simulink model "simulation_4_different_capacity"  (R2026a)
settings: Solver=VariableStepAuto  StopTime=12000
undefined symbols (not defined in the file): battery_builder_rtmsupport, gcbh
libraries: fl_lib x36, nesl_utility x18, BatteryCurrentManagement x6, Batteries_lib x6, BatteryEstimators x6
(part 1 of 2)
settings Model: Creator=dom  LastModifiedBy=dom

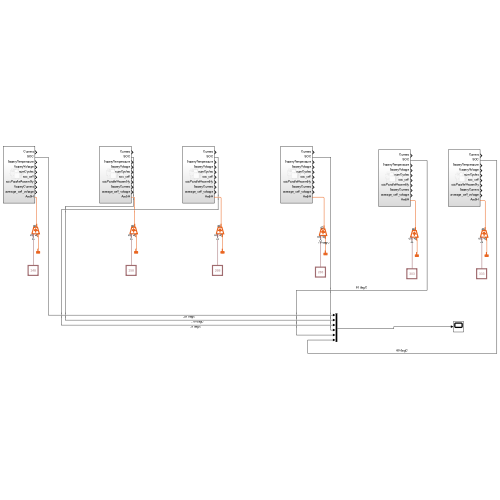
[thumbnail: Simulink's stored preview of the top-level diagram]
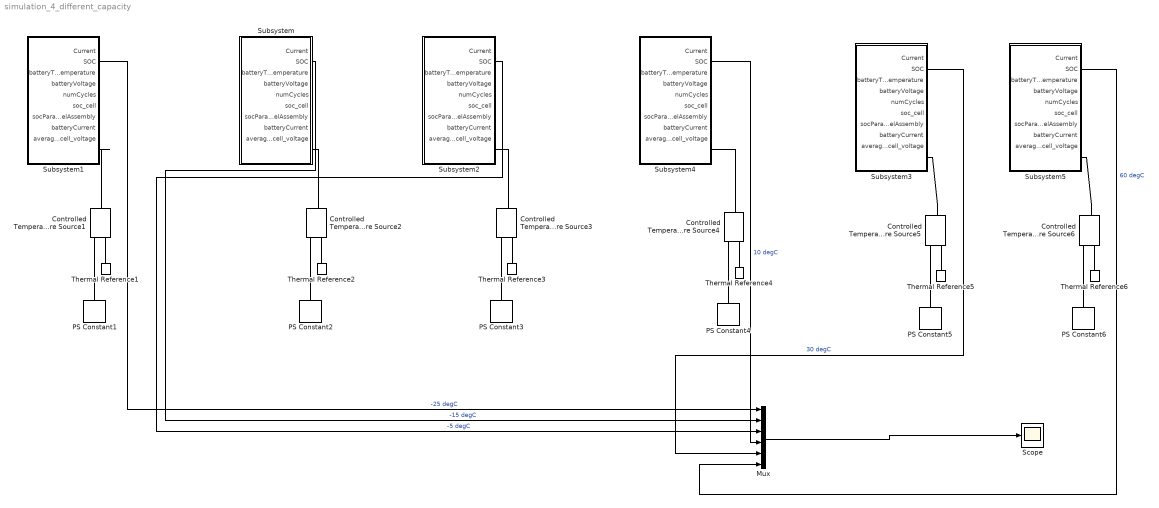
== system simulation_4_different_capacity ==
  Controlled Temperature Source{1..6} (6 alike) : fl_lib/Thermal/Thermal Sources/Controlled Temperature Source
  Mux : Mux  Inputs=6
  PS Constant1 : fl_lib/Physical Signals/Sources/PS Constant  constant=248 K
  PS Constant2 : fl_lib/Physical Signals/Sources/PS Constant  constant=258 K
  PS Constant3 : fl_lib/Physical Signals/Sources/PS Constant  constant=268 K
  PS Constant4 : fl_lib/Physical Signals/Sources/PS Constant  constant=283 K
  PS Constant5 : fl_lib/Physical Signals/Sources/PS Constant  constant=303 K
  PS Constant6 : fl_lib/Physical Signals/Sources/PS Constant  constant=333 K
  Scope : Scope
      settings: ActiveDisplayYMinimum=2.8193312500000003  ActiveDisplayYMaximum=4.3218187500000012
  Subsystem : Subsystem
  Subsystem1 : Subsystem
  Subsystem2 : Subsystem
  Subsystem3 : Subsystem
  Subsystem4 : Subsystem
  Subsystem5 : Subsystem
  Thermal Reference{1..6} (6 alike) : fl_lib/Thermal/Thermal Elements/Thermal Reference
  wires:
  Mux/1 -> Scope/1
  Subsystem1/2(SOC) -> Mux/1  "-25 degC"
  Subsystem/2(SOC) -> Mux/2  "-15 degC"
  Subsystem2/2(SOC) -> Mux/3  "-5 degC"
  Subsystem4/2(SOC) -> Mux/4  "10 degC"
  Subsystem3/2(SOC) -> Mux/5  "30 degC"
  Subsystem5/2(SOC) -> Mux/6  "60 degC"
  connections:
  PS Constant1/RConn1 -- Controlled Temperature Source1/RConn1
  Controlled Temperature Source1/RConn2 -- Thermal Reference1/LConn1
  Subsystem1/RConn1 -- Controlled Temperature Source1/LConn1
  Controlled Temperature Source2/LConn1 -- Subsystem/RConn1
  PS Constant2/RConn1 -- Controlled Temperature Source2/RConn1
  Controlled Temperature Source2/RConn2 -- Thermal Reference2/LConn1
  Controlled Temperature Source3/LConn1 -- Subsystem2/RConn1
  PS Constant3/RConn1 -- Controlled Temperature Source3/RConn1
  Controlled Temperature Source3/RConn2 -- Thermal Reference3/LConn1
  Controlled Temperature Source4/LConn1 -- Subsystem4/RConn1
  PS Constant4/RConn1 -- Controlled Temperature Source4/RConn1
  Controlled Temperature Source4/RConn2 -- Thermal Reference4/LConn1
  Controlled Temperature Source5/LConn1 -- Subsystem3/RConn1
  PS Constant5/RConn1 -- Controlled Temperature Source5/RConn1
  Controlled Temperature Source5/RConn2 -- Thermal Reference5/LConn1
  PS Constant6/RConn1 -- Controlled Temperature Source6/RConn1
  Controlled Temperature Source6/RConn2 -- Thermal Reference6/LConn1
  Controlled Temperature Source6/LConn1 -- Subsystem5/RConn1

== system simulation_4_different_capacity/Subsystem ==
  CC-CV Controller : BatteryCurrentManagement/Battery CC-CV  MinMaxFlag=off  MaxCellVoltage=4.2  Kp=100  Ki=10  Kaw=1  Kt=1  Ts=1
      settings: LibrarySourceBlock=batt_sl_lib/Current Management/Battery CC-CV
  Constant : Constant
  Constant1 : Constant  Value=10.4
  Controlled Current Source : fl_lib/Electrical/Electrical Sources/Controlled Current Source
  Current Sensor : fl_lib/Electrical/Electrical Sensors/Current Sensor
  Electrical Reference : fl_lib/Electrical/Electrical Elements/Electrical Reference
  Gain : Gain  Gain=0.5
  Gain1 : Gain  Gain=-1
  Mean : MATLAB Function  TreatAsAtomicUnit=on
  ODPC : MATLAB Function  TreatAsAtomicUnit=on
  PS-Simulink Converter : nesl_utility/PS-Simulink Converter  PhysicalDomain=network_engine_domain  SubClassName=ps_output  LeftPortType=input  RightPortType=output  PseudoPeriodic=off  Frequencies=[]  VectorFormat=inherit  Unit=inherit  AffineConversion=off
  Project_Pack : Subsystem  LoadFcn=battery_builder_rtmsupport('loadfcn',gcbh);
      settings: CopyFcn=battery_builder_rtmsupport('copyfcn',gcbh);  PreCopyFcn=battery_builder_rtmsupport('precopyfcn',gcbh);  PreDeleteFcn=battery_builder_rtmsupport('predeletefcn',gcbh);  PortSchema="{\"entries\":[{\"content\":{\"sides\":[{\"content\":{\"connectorIds\":[\"LConn1\"]},\"type\":\"ConnectorPlacement.EquallySpacedRectSide\",\"uuid\":\"76c6f046-db8e-4015-a922-00ba973faf16\"},{\"content\":{\"connectorIds\":[\"RConn1\",\"RConn2\"],\"side\":\"RIGHT\"},\"type\":\"ConnectorPlacement.EquallySpacedRectSide\",\"uuid\":\"59fdee5c-a6f4-4b44-aa6e-82d2d9418fce\"},{\"content\":{\"connectorIds\":[\"Out7\"],\"side\":\"TOP\"},\"type\":\"ConnectorPlacement.EquallySpacedRectSide\",\"uuid\":\"84b83595-cc1f-46da-a2b0-c16634a6daab\"},{\"content\":{\"connectorIds\":[\"Out1\",\"Out2\",\"Out3\",\"Out4\",\"Out5\",\"Out6\"],\"side\":\"BOTTOM\"},\"type\":\"ConnectorPlacement.EquallySpacedRectSide\",\"uuid\":\"4528fa0d-8164-4e66-baa6-2a345765de4f\"}]},\"type\":\"ConnectorPlacement.EquallySpacedConnector\",\"uuid\":\"e6fb231a-8daf-4bfc-bdc1-9175fa7a2dfd\"}],\"packageUris\":[\"http://schema.mathworks.com/mf0/Connector/R2020b\"],\"version\":\"1.0\"}"
      mask Display: image('$imagefile')
  Relay : Relay  OnSwitchValue=1  OffSwitchValue=0  OnOutputValue=0  OffOutputValue=1
  "SOC Estimator " : BatteryEstimators/SOC Estimator (Coulomb Counting)  CurrentInputPartition=off  AH=7.08  Ts=1  DataType=Inherit: auto
      settings: LibrarySourceBlock=|
      | batt_sl_lib/Estimators/SOC Estimator
      | (Coulomb Counting)
  Simulink-PS Converter1 : nesl_utility/Simulink-PS Converter  PhysicalDomain=network_engine_domain  SubClassName=ps_input  LeftPortType=input  RightPortType=output  PseudoPeriodic=off  Frequencies=[]  NoiseDistribution=none  NoiseParameters=[]  Unit=1  AffineConversion=off  FilteringAndDerivatives=provide  SimscapeFilterOrder=1  InputFilterTimeConstant=0.001  UdotUserProvided=0
  Solver Configuration : nesl_utility/Solver Configuration  PhysicalDomain=network_engine_domain  SubClassName=solver  LeftPortType=input  RightPortType=generic  Tones=[]  Harmonics=[]  SimulateNoise=off  Profile=off  UseLocalSampling=off  EnableSwitchedLinearOptims=on  FrequencyDomain=off  UseCCode=off  RelTol=0.001  AbsTol=0.001  MinStep=1e-09  ToWorkspace=off  RevertToSquareIcSolve=off  NumHomotopyIterations=100  PhasorMode=off  PhasorModeNumHarmonics=1  ConsistencySolver=NEWTON_XTOL_AFTER_FTOL  CanonicalOrdering=CANONICAL  OptimizeIntermediates=OPTIMIZED  IndexReductionMethod=DerivativeReplacement  DoDC=off  ResidualTolerance=1e-09  ConsistencyTolSource=GLOBAL  ConsistencyAbsTol=0.001  ConsistencyRelTol=0.001  ConsistencyTolFactor=0.001  UseLocalSolver=off  LocalSolverChoice=NE_BACKWARD_EULER_ADVANCER  ResolveIndetEquations=on  FunctionEvalNumThread=1  LocalSolverSampleTime=0.001  DoFixedCost=off  MaxNonlinIter=3  MaxModeIter=2  ComputeImpulses=off  ImpulseIterations=2  LinearAlgebra=auto  LinearAlgebraNumThread=0  EquationFormulation=NE_TIME_EF  DelaysMemoryBudget=1024  AutomaticFiltering=on  FilteringTimeConstant=0.001  PartitionStorageMethod=AS_NEEDED  PartitionMemoryBudget=1024  PartitionMethod=ROBUST  MultibodyUseLocalSolver=off  MultibodyLocalSolverChoice=ODE1  MultibodyLocalSolverSampleTime=0.001
  Unit Delay : UnitDelay  InitialCondition=4.2
  Unit Delay1 : UnitDelay  InitialCondition=1
  Unit Delay2 : UnitDelay  SampleTime=-1
  AmbH : PMIOPort  Side=Right
  Current : Outport
  SOC : Outport  Port=2
  batteryTemperature : Outport  Port=3
  batteryVoltage : Outport  Port=4
  numCycles : Outport  Port=5
  soc_cell : Outport  Port=6
  socParallelAssembly : Outport  Port=7
  batteryCurrent : Outport  Port=8
  average_cell_voltage : Outport  Port=9
  wires:
  Project_Pack/1(batteryTemperature) -> batteryTemperature/1  "batteryTemperature"
  CC-CV Controller/1 -> ODPC/3(CC_CV_current)
  ODPC/1(output_current) -> Simulink-PS Converter1/1  "output_current"
  Gain1/1 -> CC-CV Controller/4
  Project_Pack/3(numCycles) -> numCycles/1
  Mean/1(y) -> average_cell_voltage/1, Unit Delay/1  "average_cell_voltage"
  Project_Pack/2(batteryVoltage) -> batteryVoltage/1
  Unit Delay1/1 -> ODPC/2(SOC), Relay/1
  Unit Delay2/1 -> ODPC/1(charging_enabled)
  Constant1/1 -> Gain/1, Gain1/1  "pack_C-rate"
  Unit Delay/1 -> CC-CV Controller/2
  Project_Pack/6(batteryCurrent) -> batteryCurrent/1
  Constant/1 -> "SOC Estimator "/2
  Project_Pack/4(socCell) -> soc_cell/1  "soc_cell"
  "SOC Estimator "/1 -> SOC/1, Unit Delay1/1  "SOC"
  Project_Pack/7(vParallelAssembly) -> Mean/1(u)
  PS-Simulink Converter/1 -> Current/1, "SOC Estimator "/1
  Gain/1 -> CC-CV Controller/3
  Relay/1 -> Unit Delay2/1, CC-CV Controller/1  "charging_enabled"
  Project_Pack/5(socParallelAssembly) -> socParallelAssembly/1
  connections:
  Project_Pack/RConn1 -- AmbH/RConn1
  Controlled Current Source/LConn1 -- Project_Pack/LConn1
  Simulink-PS Converter1/RConn1 -- Controlled Current Source/RConn1
  Project_Pack/RConn2 -- Solver Configuration/RConn1 -- Current Sensor/LConn1 -- Electrical Reference/LConn1
  Current Sensor/RConn1 -- PS-Simulink Converter/LConn1
  Current Sensor/RConn2 -- Controlled Current Source/RConn2

== system simulation_4_different_capacity/Subsystem1 ==
  CC-CV Controller : BatteryCurrentManagement/Battery CC-CV  MinMaxFlag=off  MaxCellVoltage=4.2  Kp=100  Ki=10  Kaw=1  Kt=1  Ts=1
      settings: LibrarySourceBlock=batt_sl_lib/Current Management/Battery CC-CV
  Constant : Constant
  Constant1 : Constant  Value=10.4
  Controlled Current Source : fl_lib/Electrical/Electrical Sources/Controlled Current Source
  Current Sensor : fl_lib/Electrical/Electrical Sensors/Current Sensor
  Electrical Reference : fl_lib/Electrical/Electrical Elements/Electrical Reference
  Gain : Gain  Gain=0.5
  Gain1 : Gain  Gain=-1
  Mean : MATLAB Function  TreatAsAtomicUnit=on
  ODPC : MATLAB Function  TreatAsAtomicUnit=on
  PS-Simulink Converter : nesl_utility/PS-Simulink Converter  PhysicalDomain=network_engine_domain  SubClassName=ps_output  LeftPortType=input  RightPortType=output  PseudoPeriodic=off  Frequencies=[]  VectorFormat=inherit  Unit=inherit  AffineConversion=off
  Project_Pack : Subsystem  LoadFcn=battery_builder_rtmsupport('loadfcn',gcbh);
      settings: CopyFcn=battery_builder_rtmsupport('copyfcn',gcbh);  PreCopyFcn=battery_builder_rtmsupport('precopyfcn',gcbh);  PreDeleteFcn=battery_builder_rtmsupport('predeletefcn',gcbh);  PortSchema="{\"entries\":[{\"content\":{\"sides\":[{\"content\":{\"connectorIds\":[\"LConn1\"]},\"type\":\"ConnectorPlacement.EquallySpacedRectSide\",\"uuid\":\"76c6f046-db8e-4015-a922-00ba973faf16\"},{\"content\":{\"connectorIds\":[\"RConn1\",\"RConn2\"],\"side\":\"RIGHT\"},\"type\":\"ConnectorPlacement.EquallySpacedRectSide\",\"uuid\":\"59fdee5c-a6f4-4b44-aa6e-82d2d9418fce\"},{\"content\":{\"connectorIds\":[\"Out7\"],\"side\":\"TOP\"},\"type\":\"ConnectorPlacement.EquallySpacedRectSide\",\"uuid\":\"84b83595-cc1f-46da-a2b0-c16634a6daab\"},{\"content\":{\"connectorIds\":[\"Out1\",\"Out2\",\"Out3\",\"Out4\",\"Out5\",\"Out6\"],\"side\":\"BOTTOM\"},\"type\":\"ConnectorPlacement.EquallySpacedRectSide\",\"uuid\":\"4528fa0d-8164-4e66-baa6-2a345765de4f\"}]},\"type\":\"ConnectorPlacement.EquallySpacedConnector\",\"uuid\":\"e6fb231a-8daf-4bfc-bdc1-9175fa7a2dfd\"}],\"packageUris\":[\"http://schema.mathworks.com/mf0/Connector/R2020b\"],\"version\":\"1.0\"}"
      mask Display: image('$imagefile')
  Relay : Relay  OnSwitchValue=1  OffSwitchValue=0  OnOutputValue=0  OffOutputValue=1
  "SOC Estimator " : BatteryEstimators/SOC Estimator (Coulomb Counting)  CurrentInputPartition=off  AH=4.2  Ts=1  DataType=Inherit: auto
      settings: LibrarySourceBlock=|
      | batt_sl_lib/Estimators/SOC Estimator
      | (Coulomb Counting)
  Simulink-PS Converter1 : nesl_utility/Simulink-PS Converter  PhysicalDomain=network_engine_domain  SubClassName=ps_input  LeftPortType=input  RightPortType=output  PseudoPeriodic=off  Frequencies=[]  NoiseDistribution=none  NoiseParameters=[]  Unit=1  AffineConversion=off  FilteringAndDerivatives=provide  SimscapeFilterOrder=1  InputFilterTimeConstant=0.001  UdotUserProvided=0
  Solver Configuration : nesl_utility/Solver Configuration  PhysicalDomain=network_engine_domain  SubClassName=solver  LeftPortType=input  RightPortType=generic  Tones=[]  Harmonics=[]  SimulateNoise=off  Profile=off  UseLocalSampling=off  EnableSwitchedLinearOptims=on  FrequencyDomain=off  UseCCode=off  RelTol=0.001  AbsTol=0.001  MinStep=1e-09  ToWorkspace=off  RevertToSquareIcSolve=off  NumHomotopyIterations=100  PhasorMode=off  PhasorModeNumHarmonics=1  ConsistencySolver=NEWTON_XTOL_AFTER_FTOL  CanonicalOrdering=CANONICAL  OptimizeIntermediates=OPTIMIZED  IndexReductionMethod=DerivativeReplacement  DoDC=off  ResidualTolerance=1e-09  ConsistencyTolSource=GLOBAL  ConsistencyAbsTol=0.001  ConsistencyRelTol=0.001  ConsistencyTolFactor=0.001  UseLocalSolver=off  LocalSolverChoice=NE_BACKWARD_EULER_ADVANCER  ResolveIndetEquations=on  FunctionEvalNumThread=1  LocalSolverSampleTime=0.001  DoFixedCost=off  MaxNonlinIter=3  MaxModeIter=2  ComputeImpulses=off  ImpulseIterations=2  LinearAlgebra=auto  LinearAlgebraNumThread=0  EquationFormulation=NE_TIME_EF  DelaysMemoryBudget=1024  AutomaticFiltering=on  FilteringTimeConstant=0.001  PartitionStorageMethod=AS_NEEDED  PartitionMemoryBudget=1024  PartitionMethod=ROBUST  MultibodyUseLocalSolver=off  MultibodyLocalSolverChoice=ODE1  MultibodyLocalSolverSampleTime=0.001
  Unit Delay : UnitDelay  InitialCondition=4.2
  Unit Delay1 : UnitDelay  InitialCondition=1
  Unit Delay2 : UnitDelay  SampleTime=-1
  AmbH : PMIOPort  Side=Right
  Current : Outport
  SOC : Outport  Port=2
  batteryTemperature : Outport  Port=3
  batteryVoltage : Outport  Port=4
  numCycles : Outport  Port=5
  soc_cell : Outport  Port=6
  socParallelAssembly : Outport  Port=7
  batteryCurrent : Outport  Port=8
  average_cell_voltage : Outport  Port=9
  wires:
  Project_Pack/1(batteryTemperature) -> batteryTemperature/1  "batteryTemperature"
  CC-CV Controller/1 -> ODPC/3(CC_CV_current)
  ODPC/1(output_current) -> Simulink-PS Converter1/1  "output_current"
  Gain1/1 -> CC-CV Controller/4
  Project_Pack/3(numCycles) -> numCycles/1
  Mean/1(y) -> average_cell_voltage/1, Unit Delay/1  "average_cell_voltage"
  Project_Pack/2(batteryVoltage) -> batteryVoltage/1
  Unit Delay1/1 -> ODPC/2(SOC), Relay/1
  Unit Delay2/1 -> ODPC/1(charging_enabled)
  Constant1/1 -> Gain/1, Gain1/1  "pack_C-rate"
  Unit Delay/1 -> CC-CV Controller/2
  Project_Pack/6(batteryCurrent) -> batteryCurrent/1
  Constant/1 -> "SOC Estimator "/2
  Project_Pack/4(socCell) -> soc_cell/1  "soc_cell"
  "SOC Estimator "/1 -> SOC/1, Unit Delay1/1  "SOC"
  Project_Pack/7(vParallelAssembly) -> Mean/1(u)
  PS-Simulink Converter/1 -> Current/1, "SOC Estimator "/1
  Gain/1 -> CC-CV Controller/3
  Relay/1 -> Unit Delay2/1, CC-CV Controller/1  "charging_enabled"
  Project_Pack/5(socParallelAssembly) -> socParallelAssembly/1
  connections:
  Project_Pack/RConn1 -- AmbH/RConn1
  Controlled Current Source/LConn1 -- Project_Pack/LConn1
  Simulink-PS Converter1/RConn1 -- Controlled Current Source/RConn1
  Project_Pack/RConn2 -- Solver Configuration/RConn1 -- Current Sensor/LConn1 -- Electrical Reference/LConn1
  Current Sensor/RConn1 -- PS-Simulink Converter/LConn1
  Current Sensor/RConn2 -- Controlled Current Source/RConn2

== system simulation_4_different_capacity/Subsystem2 ==
  CC-CV Controller : BatteryCurrentManagement/Battery CC-CV  MinMaxFlag=off  MaxCellVoltage=4.2  Kp=100  Ki=10  Kaw=1  Kt=1  Ts=1
      settings: LibrarySourceBlock=batt_sl_lib/Current Management/Battery CC-CV
  Constant : Constant
  Constant1 : Constant  Value=10.4
  Controlled Current Source : fl_lib/Electrical/Electrical Sources/Controlled Current Source
  Current Sensor : fl_lib/Electrical/Electrical Sensors/Current Sensor
  Electrical Reference : fl_lib/Electrical/Electrical Elements/Electrical Reference
  Gain : Gain  Gain=0.5
  Gain1 : Gain  Gain=-1
  Mean : MATLAB Function  TreatAsAtomicUnit=on
  ODPC : MATLAB Function  TreatAsAtomicUnit=on
  PS-Simulink Converter : nesl_utility/PS-Simulink Converter  PhysicalDomain=network_engine_domain  SubClassName=ps_output  LeftPortType=input  RightPortType=output  PseudoPeriodic=off  Frequencies=[]  VectorFormat=inherit  Unit=inherit  AffineConversion=off
  Project_Pack : Subsystem  LoadFcn=battery_builder_rtmsupport('loadfcn',gcbh);
      settings: CopyFcn=battery_builder_rtmsupport('copyfcn',gcbh);  PreCopyFcn=battery_builder_rtmsupport('precopyfcn',gcbh);  PreDeleteFcn=battery_builder_rtmsupport('predeletefcn',gcbh);  PortSchema="{\"entries\":[{\"content\":{\"sides\":[{\"content\":{\"connectorIds\":[\"LConn1\"]},\"type\":\"ConnectorPlacement.EquallySpacedRectSide\",\"uuid\":\"76c6f046-db8e-4015-a922-00ba973faf16\"},{\"content\":{\"connectorIds\":[\"RConn1\",\"RConn2\"],\"side\":\"RIGHT\"},\"type\":\"ConnectorPlacement.EquallySpacedRectSide\",\"uuid\":\"59fdee5c-a6f4-4b44-aa6e-82d2d9418fce\"},{\"content\":{\"connectorIds\":[\"Out7\"],\"side\":\"TOP\"},\"type\":\"ConnectorPlacement.EquallySpacedRectSide\",\"uuid\":\"84b83595-cc1f-46da-a2b0-c16634a6daab\"},{\"content\":{\"connectorIds\":[\"Out1\",\"Out2\",\"Out3\",\"Out4\",\"Out5\",\"Out6\"],\"side\":\"BOTTOM\"},\"type\":\"ConnectorPlacement.EquallySpacedRectSide\",\"uuid\":\"4528fa0d-8164-4e66-baa6-2a345765de4f\"}]},\"type\":\"ConnectorPlacement.EquallySpacedConnector\",\"uuid\":\"e6fb231a-8daf-4bfc-bdc1-9175fa7a2dfd\"}],\"packageUris\":[\"http://schema.mathworks.com/mf0/Connector/R2020b\"],\"version\":\"1.0\"}"
      mask Display: image('$imagefile')
  Relay : Relay  OnSwitchValue=1  OffSwitchValue=0  OnOutputValue=0  OffOutputValue=1
  "SOC Estimator " : BatteryEstimators/SOC Estimator (Coulomb Counting)  CurrentInputPartition=off  AH=9.20  Ts=1  DataType=Inherit: auto
      settings: LibrarySourceBlock=|
      | batt_sl_lib/Estimators/SOC Estimator
      | (Coulomb Counting)
  Simulink-PS Converter1 : nesl_utility/Simulink-PS Converter  PhysicalDomain=network_engine_domain  SubClassName=ps_input  LeftPortType=input  RightPortType=output  PseudoPeriodic=off  Frequencies=[]  NoiseDistribution=none  NoiseParameters=[]  Unit=1  AffineConversion=off  FilteringAndDerivatives=provide  SimscapeFilterOrder=1  InputFilterTimeConstant=0.001  UdotUserProvided=0
  Solver Configuration : nesl_utility/Solver Configuration  PhysicalDomain=network_engine_domain  SubClassName=solver  LeftPortType=input  RightPortType=generic  Tones=[]  Harmonics=[]  SimulateNoise=off  Profile=off  UseLocalSampling=off  EnableSwitchedLinearOptims=on  FrequencyDomain=off  UseCCode=off  RelTol=0.001  AbsTol=0.001  MinStep=1e-09  ToWorkspace=off  RevertToSquareIcSolve=off  NumHomotopyIterations=100  PhasorMode=off  PhasorModeNumHarmonics=1  ConsistencySolver=NEWTON_XTOL_AFTER_FTOL  CanonicalOrdering=CANONICAL  OptimizeIntermediates=OPTIMIZED  IndexReductionMethod=DerivativeReplacement  DoDC=off  ResidualTolerance=1e-09  ConsistencyTolSource=GLOBAL  ConsistencyAbsTol=0.001  ConsistencyRelTol=0.001  ConsistencyTolFactor=0.001  UseLocalSolver=off  LocalSolverChoice=NE_BACKWARD_EULER_ADVANCER  ResolveIndetEquations=on  FunctionEvalNumThread=1  LocalSolverSampleTime=0.001  DoFixedCost=off  MaxNonlinIter=3  MaxModeIter=2  ComputeImpulses=off  ImpulseIterations=2  LinearAlgebra=auto  LinearAlgebraNumThread=0  EquationFormulation=NE_TIME_EF  DelaysMemoryBudget=1024  AutomaticFiltering=on  FilteringTimeConstant=0.001  PartitionStorageMethod=AS_NEEDED  PartitionMemoryBudget=1024  PartitionMethod=ROBUST  MultibodyUseLocalSolver=off  MultibodyLocalSolverChoice=ODE1  MultibodyLocalSolverSampleTime=0.001
  Unit Delay : UnitDelay  InitialCondition=4.2
  Unit Delay1 : UnitDelay  InitialCondition=1
  Unit Delay2 : UnitDelay  SampleTime=-1
  AmbH : PMIOPort  Side=Right
  Current : Outport
  SOC : Outport  Port=2
  batteryTemperature : Outport  Port=3
  batteryVoltage : Outport  Port=4
  numCycles : Outport  Port=5
  soc_cell : Outport  Port=6
  socParallelAssembly : Outport  Port=7
  batteryCurrent : Outport  Port=8
  average_cell_voltage : Outport  Port=9
  wires:
  Project_Pack/1(batteryTemperature) -> batteryTemperature/1  "batteryTemperature"
  CC-CV Controller/1 -> ODPC/3(CC_CV_current)
  ODPC/1(output_current) -> Simulink-PS Converter1/1  "output_current"
  Gain1/1 -> CC-CV Controller/4
  Project_Pack/3(numCycles) -> numCycles/1
  Mean/1(y) -> average_cell_voltage/1, Unit Delay/1  "average_cell_voltage"
  Project_Pack/2(batteryVoltage) -> batteryVoltage/1
  Unit Delay1/1 -> ODPC/2(SOC), Relay/1
  Unit Delay2/1 -> ODPC/1(charging_enabled)
  Constant1/1 -> Gain/1, Gain1/1  "pack_C-rate"
  Unit Delay/1 -> CC-CV Controller/2
  Project_Pack/6(batteryCurrent) -> batteryCurrent/1
  Constant/1 -> "SOC Estimator "/2
  Project_Pack/4(socCell) -> soc_cell/1  "soc_cell"
  "SOC Estimator "/1 -> SOC/1, Unit Delay1/1  "SOC"
  Project_Pack/7(vParallelAssembly) -> Mean/1(u)
  PS-Simulink Converter/1 -> Current/1, "SOC Estimator "/1
  Gain/1 -> CC-CV Controller/3
  Relay/1 -> Unit Delay2/1, CC-CV Controller/1  "charging_enabled"
  Project_Pack/5(socParallelAssembly) -> socParallelAssembly/1
  connections:
  Project_Pack/RConn1 -- AmbH/RConn1
  Controlled Current Source/LConn1 -- Project_Pack/LConn1
  Simulink-PS Converter1/RConn1 -- Controlled Current Source/RConn1
  Project_Pack/RConn2 -- Solver Configuration/RConn1 -- Current Sensor/LConn1 -- Electrical Reference/LConn1
  Current Sensor/RConn1 -- PS-Simulink Converter/LConn1
  Current Sensor/RConn2 -- Controlled Current Source/RConn2

== system simulation_4_different_capacity/Subsystem3 ==
  CC-CV Controller : BatteryCurrentManagement/Battery CC-CV  MinMaxFlag=off  MaxCellVoltage=4.2  Kp=100  Ki=10  Kaw=1  Kt=1  Ts=1
      settings: LibrarySourceBlock=batt_sl_lib/Current Management/Battery CC-CV
  Constant : Constant
  Constant1 : Constant  Value=10.4
  Controlled Current Source : fl_lib/Electrical/Electrical Sources/Controlled Current Source
  Current Sensor : fl_lib/Electrical/Electrical Sensors/Current Sensor
  Electrical Reference : fl_lib/Electrical/Electrical Elements/Electrical Reference
  Gain : Gain  Gain=0.5
  Gain1 : Gain  Gain=-1
  Mean : MATLAB Function  TreatAsAtomicUnit=on
  ODPC : MATLAB Function  TreatAsAtomicUnit=on
  PS-Simulink Converter : nesl_utility/PS-Simulink Converter  PhysicalDomain=network_engine_domain  SubClassName=ps_output  LeftPortType=input  RightPortType=output  PseudoPeriodic=off  Frequencies=[]  VectorFormat=inherit  Unit=inherit  AffineConversion=off
  Project_Pack : Subsystem  LoadFcn=battery_builder_rtmsupport('loadfcn',gcbh);
      settings: CopyFcn=battery_builder_rtmsupport('copyfcn',gcbh);  PreCopyFcn=battery_builder_rtmsupport('precopyfcn',gcbh);  PreDeleteFcn=battery_builder_rtmsupport('predeletefcn',gcbh);  PortSchema="{\"entries\":[{\"content\":{\"sides\":[{\"content\":{\"connectorIds\":[\"LConn1\"]},\"type\":\"ConnectorPlacement.EquallySpacedRectSide\",\"uuid\":\"76c6f046-db8e-4015-a922-00ba973faf16\"},{\"content\":{\"connectorIds\":[\"RConn1\",\"RConn2\"],\"side\":\"RIGHT\"},\"type\":\"ConnectorPlacement.EquallySpacedRectSide\",\"uuid\":\"59fdee5c-a6f4-4b44-aa6e-82d2d9418fce\"},{\"content\":{\"connectorIds\":[\"Out7\"],\"side\":\"TOP\"},\"type\":\"ConnectorPlacement.EquallySpacedRectSide\",\"uuid\":\"84b83595-cc1f-46da-a2b0-c16634a6daab\"},{\"content\":{\"connectorIds\":[\"Out1\",\"Out2\",\"Out3\",\"Out4\",\"Out5\",\"Out6\"],\"side\":\"BOTTOM\"},\"type\":\"ConnectorPlacement.EquallySpacedRectSide\",\"uuid\":\"4528fa0d-8164-4e66-baa6-2a345765de4f\"}]},\"type\":\"ConnectorPlacement.EquallySpacedConnector\",\"uuid\":\"e6fb231a-8daf-4bfc-bdc1-9175fa7a2dfd\"}],\"packageUris\":[\"http://schema.mathworks.com/mf0/Connector/R2020b\"],\"version\":\"1.0\"}"
      mask Display: image('$imagefile')
  Relay : Relay  OnSwitchValue=1  OffSwitchValue=0  OnOutputValue=0  OffOutputValue=1
  "SOC Estimator " : BatteryEstimators/SOC Estimator (Coulomb Counting)  CurrentInputPartition=off  AH=10.4  Ts=1  DataType=Inherit: auto
      settings: LibrarySourceBlock=|
      | batt_sl_lib/Estimators/SOC Estimator
      | (Coulomb Counting)
  Simulink-PS Converter1 : nesl_utility/Simulink-PS Converter  PhysicalDomain=network_engine_domain  SubClassName=ps_input  LeftPortType=input  RightPortType=output  PseudoPeriodic=off  Frequencies=[]  NoiseDistribution=none  NoiseParameters=[]  Unit=1  AffineConversion=off  FilteringAndDerivatives=provide  SimscapeFilterOrder=1  InputFilterTimeConstant=0.001  UdotUserProvided=0
  Solver Configuration : nesl_utility/Solver Configuration  PhysicalDomain=network_engine_domain  SubClassName=solver  LeftPortType=input  RightPortType=generic  Tones=[]  Harmonics=[]  SimulateNoise=off  Profile=off  UseLocalSampling=off  EnableSwitchedLinearOptims=on  FrequencyDomain=off  UseCCode=off  RelTol=0.001  AbsTol=0.001  MinStep=1e-09  ToWorkspace=off  RevertToSquareIcSolve=off  NumHomotopyIterations=100  PhasorMode=off  PhasorModeNumHarmonics=1  ConsistencySolver=NEWTON_XTOL_AFTER_FTOL  CanonicalOrdering=CANONICAL  OptimizeIntermediates=OPTIMIZED  IndexReductionMethod=DerivativeReplacement  DoDC=off  ResidualTolerance=1e-09  ConsistencyTolSource=GLOBAL  ConsistencyAbsTol=0.001  ConsistencyRelTol=0.001  ConsistencyTolFactor=0.001  UseLocalSolver=off  LocalSolverChoice=NE_BACKWARD_EULER_ADVANCER  ResolveIndetEquations=on  FunctionEvalNumThread=1  LocalSolverSampleTime=0.001  DoFixedCost=off  MaxNonlinIter=3  MaxModeIter=2  ComputeImpulses=off  ImpulseIterations=2  LinearAlgebra=auto  LinearAlgebraNumThread=0  EquationFormulation=NE_TIME_EF  DelaysMemoryBudget=1024  AutomaticFiltering=on  FilteringTimeConstant=0.001  PartitionStorageMethod=AS_NEEDED  PartitionMemoryBudget=1024  PartitionMethod=ROBUST  MultibodyUseLocalSolver=off  MultibodyLocalSolverChoice=ODE1  MultibodyLocalSolverSampleTime=0.001
  Unit Delay : UnitDelay  InitialCondition=4.2
  Unit Delay1 : UnitDelay  InitialCondition=1
  Unit Delay2 : UnitDelay  SampleTime=-1
  AmbH : PMIOPort  Side=Right
  Current : Outport
  SOC : Outport  Port=2
  batteryTemperature : Outport  Port=3
  batteryVoltage : Outport  Port=4
  numCycles : Outport  Port=5
  soc_cell : Outport  Port=6
  socParallelAssembly : Outport  Port=7
  batteryCurrent : Outport  Port=8
  average_cell_voltage : Outport  Port=9
  wires:
  Project_Pack/1(batteryTemperature) -> batteryTemperature/1  "batteryTemperature"
  CC-CV Controller/1 -> ODPC/3(CC_CV_current)
  ODPC/1(output_current) -> Simulink-PS Converter1/1  "output_current"
  Gain1/1 -> CC-CV Controller/4
  Project_Pack/3(numCycles) -> numCycles/1
  Mean/1(y) -> average_cell_voltage/1, Unit Delay/1  "average_cell_voltage"
  Project_Pack/2(batteryVoltage) -> batteryVoltage/1
  Unit Delay1/1 -> ODPC/2(SOC), Relay/1
  Unit Delay2/1 -> ODPC/1(charging_enabled)
  Constant1/1 -> Gain/1, Gain1/1  "pack_C-rate"
  Unit Delay/1 -> CC-CV Controller/2
  Project_Pack/6(batteryCurrent) -> batteryCurrent/1
  Constant/1 -> "SOC Estimator "/2
  Project_Pack/4(socCell) -> soc_cell/1  "soc_cell"
  "SOC Estimator "/1 -> SOC/1, Unit Delay1/1  "SOC"
  Project_Pack/7(vParallelAssembly) -> Mean/1(u)
  PS-Simulink Converter/1 -> Current/1, "SOC Estimator "/1
  Gain/1 -> CC-CV Controller/3
  Relay/1 -> Unit Delay2/1, CC-CV Controller/1  "charging_enabled"
  Project_Pack/5(socParallelAssembly) -> socParallelAssembly/1
  connections:
  Project_Pack/RConn1 -- AmbH/RConn1
  Controlled Current Source/LConn1 -- Project_Pack/LConn1
  Simulink-PS Converter1/RConn1 -- Controlled Current Source/RConn1
  Project_Pack/RConn2 -- Solver Configuration/RConn1 -- Current Sensor/LConn1 -- Electrical Reference/LConn1
  Current Sensor/RConn1 -- PS-Simulink Converter/LConn1
  Current Sensor/RConn2 -- Controlled Current Source/RConn2

== system simulation_4_different_capacity/Subsystem4 ==
  CC-CV Controller : BatteryCurrentManagement/Battery CC-CV  MinMaxFlag=off  MaxCellVoltage=4.2  Kp=100  Ki=10  Kaw=1  Kt=1  Ts=1
      settings: LibrarySourceBlock=batt_sl_lib/Current Management/Battery CC-CV
  Constant : Constant
  Constant1 : Constant  Value=10.4
  Controlled Current Source : fl_lib/Electrical/Electrical Sources/Controlled Current Source
  Current Sensor : fl_lib/Electrical/Electrical Sensors/Current Sensor
  Electrical Reference : fl_lib/Electrical/Electrical Elements/Electrical Reference
  Gain : Gain  Gain=0.5
  Gain1 : Gain  Gain=-1
  Mean : MATLAB Function  TreatAsAtomicUnit=on
  ODPC : MATLAB Function  TreatAsAtomicUnit=on
  PS-Simulink Converter : nesl_utility/PS-Simulink Converter  PhysicalDomain=network_engine_domain  SubClassName=ps_output  LeftPortType=input  RightPortType=output  PseudoPeriodic=off  Frequencies=[]  VectorFormat=inherit  Unit=inherit  AffineConversion=off
  Project_Pack : Subsystem  LoadFcn=battery_builder_rtmsupport('loadfcn',gcbh);
      settings: CopyFcn=battery_builder_rtmsupport('copyfcn',gcbh);  PreCopyFcn=battery_builder_rtmsupport('precopyfcn',gcbh);  PreDeleteFcn=battery_builder_rtmsupport('predeletefcn',gcbh);  PortSchema="{\"entries\":[{\"content\":{\"sides\":[{\"content\":{\"connectorIds\":[\"LConn1\"]},\"type\":\"ConnectorPlacement.EquallySpacedRectSide\",\"uuid\":\"76c6f046-db8e-4015-a922-00ba973faf16\"},{\"content\":{\"connectorIds\":[\"RConn1\",\"RConn2\"],\"side\":\"RIGHT\"},\"type\":\"ConnectorPlacement.EquallySpacedRectSide\",\"uuid\":\"59fdee5c-a6f4-4b44-aa6e-82d2d9418fce\"},{\"content\":{\"connectorIds\":[\"Out7\"],\"side\":\"TOP\"},\"type\":\"ConnectorPlacement.EquallySpacedRectSide\",\"uuid\":\"84b83595-cc1f-46da-a2b0-c16634a6daab\"},{\"content\":{\"connectorIds\":[\"Out1\",\"Out2\",\"Out3\",\"Out4\",\"Out5\",\"Out6\"],\"side\":\"BOTTOM\"},\"type\":\"ConnectorPlacement.EquallySpacedRectSide\",\"uuid\":\"4528fa0d-8164-4e66-baa6-2a345765de4f\"}]},\"type\":\"ConnectorPlacement.EquallySpacedConnector\",\"uuid\":\"e6fb231a-8daf-4bfc-bdc1-9175fa7a2dfd\"}],\"packageUris\":[\"http://schema.mathworks.com/mf0/Connector/R2020b\"],\"version\":\"1.0\"}"
      mask Display: image('$imagefile')
  Relay : Relay  OnSwitchValue=1  OffSwitchValue=0  OnOutputValue=0  OffOutputValue=1
  "SOC Estimator " : BatteryEstimators/SOC Estimator (Coulomb Counting)  CurrentInputPartition=off  AH=10.0  Ts=1  DataType=Inherit: auto
      settings: LibrarySourceBlock=|
      | batt_sl_lib/Estimators/SOC Estimator
      | (Coulomb Counting)
  Simulink-PS Converter1 : nesl_utility/Simulink-PS Converter  PhysicalDomain=network_engine_domain  SubClassName=ps_input  LeftPortType=input  RightPortType=output  PseudoPeriodic=off  Frequencies=[]  NoiseDistribution=none  NoiseParameters=[]  Unit=1  AffineConversion=off  FilteringAndDerivatives=provide  SimscapeFilterOrder=1  InputFilterTimeConstant=0.001  UdotUserProvided=0
  Solver Configuration : nesl_utility/Solver Configuration  PhysicalDomain=network_engine_domain  SubClassName=solver  LeftPortType=input  RightPortType=generic  Tones=[]  Harmonics=[]  SimulateNoise=off  Profile=off  UseLocalSampling=off  EnableSwitchedLinearOptims=on  FrequencyDomain=off  UseCCode=off  RelTol=0.001  AbsTol=0.001  MinStep=1e-09  ToWorkspace=off  RevertToSquareIcSolve=off  NumHomotopyIterations=100  PhasorMode=off  PhasorModeNumHarmonics=1  ConsistencySolver=NEWTON_XTOL_AFTER_FTOL  CanonicalOrdering=CANONICAL  OptimizeIntermediates=OPTIMIZED  IndexReductionMethod=DerivativeReplacement  DoDC=off  ResidualTolerance=1e-09  ConsistencyTolSource=GLOBAL  ConsistencyAbsTol=0.001  ConsistencyRelTol=0.001  ConsistencyTolFactor=0.001  UseLocalSolver=off  LocalSolverChoice=NE_BACKWARD_EULER_ADVANCER  ResolveIndetEquations=on  FunctionEvalNumThread=1  LocalSolverSampleTime=0.001  DoFixedCost=off  MaxNonlinIter=3  MaxModeIter=2  ComputeImpulses=off  ImpulseIterations=2  LinearAlgebra=auto  LinearAlgebraNumThread=0  EquationFormulation=NE_TIME_EF  DelaysMemoryBudget=1024  AutomaticFiltering=on  FilteringTimeConstant=0.001  PartitionStorageMethod=AS_NEEDED  PartitionMemoryBudget=1024  PartitionMethod=ROBUST  MultibodyUseLocalSolver=off  MultibodyLocalSolverChoice=ODE1  MultibodyLocalSolverSampleTime=0.001
  Unit Delay : UnitDelay  InitialCondition=4.2
  Unit Delay1 : UnitDelay  InitialCondition=1
  Unit Delay2 : UnitDelay  SampleTime=-1
  AmbH : PMIOPort  Side=Right
  Current : Outport
  SOC : Outport  Port=2
  batteryTemperature : Outport  Port=3
  batteryVoltage : Outport  Port=4
  numCycles : Outport  Port=5
  soc_cell : Outport  Port=6
  socParallelAssembly : Outport  Port=7
  batteryCurrent : Outport  Port=8
  average_cell_voltage : Outport  Port=9
  wires:
  Project_Pack/1(batteryTemperature) -> batteryTemperature/1  "batteryTemperature"
  CC-CV Controller/1 -> ODPC/3(CC_CV_current)
  ODPC/1(output_current) -> Simulink-PS Converter1/1  "output_current"
  Gain1/1 -> CC-CV Controller/4
  Project_Pack/3(numCycles) -> numCycles/1
  Mean/1(y) -> average_cell_voltage/1, Unit Delay/1  "average_cell_voltage"
  Project_Pack/2(batteryVoltage) -> batteryVoltage/1
  Unit Delay1/1 -> ODPC/2(SOC), Relay/1
  Unit Delay2/1 -> ODPC/1(charging_enabled)
  Constant1/1 -> Gain/1, Gain1/1  "pack_C-rate"
  Unit Delay/1 -> CC-CV Controller/2
  Project_Pack/6(batteryCurrent) -> batteryCurrent/1
  Constant/1 -> "SOC Estimator "/2
  Project_Pack/4(socCell) -> soc_cell/1  "soc_cell"
  "SOC Estimator "/1 -> SOC/1, Unit Delay1/1  "SOC"
  Project_Pack/7(vParallelAssembly) -> Mean/1(u)
  PS-Simulink Converter/1 -> Current/1, "SOC Estimator "/1
  Gain/1 -> CC-CV Controller/3
  Relay/1 -> Unit Delay2/1, CC-CV Controller/1  "charging_enabled"
  Project_Pack/5(socParallelAssembly) -> socParallelAssembly/1
  connections:
  Project_Pack/RConn1 -- AmbH/RConn1
  Controlled Current Source/LConn1 -- Project_Pack/LConn1
  Simulink-PS Converter1/RConn1 -- Controlled Current Source/RConn1
  Project_Pack/RConn2 -- Solver Configuration/RConn1 -- Current Sensor/LConn1 -- Electrical Reference/LConn1
  Current Sensor/RConn1 -- PS-Simulink Converter/LConn1
  Current Sensor/RConn2 -- Controlled Current Source/RConn2

== system simulation_4_different_capacity/Subsystem5 ==
  CC-CV Controller : BatteryCurrentManagement/Battery CC-CV  MinMaxFlag=off  MaxCellVoltage=4.2  Kp=100  Ki=10  Kaw=1  Kt=1  Ts=1
      settings: LibrarySourceBlock=batt_sl_lib/Current Management/Battery CC-CV
  Constant : Constant
  Constant1 : Constant  Value=10.4
  Controlled Current Source : fl_lib/Electrical/Electrical Sources/Controlled Current Source
  Current Sensor : fl_lib/Electrical/Electrical Sensors/Current Sensor
  Electrical Reference : fl_lib/Electrical/Electrical Elements/Electrical Reference
  Gain : Gain  Gain=0.5
  Gain1 : Gain  Gain=-1
  Mean : MATLAB Function  TreatAsAtomicUnit=on
  ODPC : MATLAB Function  TreatAsAtomicUnit=on
  PS-Simulink Converter : nesl_utility/PS-Simulink Converter  PhysicalDomain=network_engine_domain  SubClassName=ps_output  LeftPortType=input  RightPortType=output  PseudoPeriodic=off  Frequencies=[]  VectorFormat=inherit  Unit=inherit  AffineConversion=off
  Project_Pack : Subsystem  LoadFcn=battery_builder_rtmsupport('loadfcn',gcbh);
      settings: CopyFcn=battery_builder_rtmsupport('copyfcn',gcbh);  PreCopyFcn=battery_builder_rtmsupport('precopyfcn',gcbh);  PreDeleteFcn=battery_builder_rtmsupport('predeletefcn',gcbh);  PortSchema="{\"entries\":[{\"content\":{\"sides\":[{\"content\":{\"connectorIds\":[\"LConn1\"]},\"type\":\"ConnectorPlacement.EquallySpacedRectSide\",\"uuid\":\"76c6f046-db8e-4015-a922-00ba973faf16\"},{\"content\":{\"connectorIds\":[\"RConn1\",\"RConn2\"],\"side\":\"RIGHT\"},\"type\":\"ConnectorPlacement.EquallySpacedRectSide\",\"uuid\":\"59fdee5c-a6f4-4b44-aa6e-82d2d9418fce\"},{\"content\":{\"connectorIds\":[\"Out7\"],\"side\":\"TOP\"},\"type\":\"ConnectorPlacement.EquallySpacedRectSide\",\"uuid\":\"84b83595-cc1f-46da-a2b0-c16634a6daab\"},{\"content\":{\"connectorIds\":[\"Out1\",\"Out2\",\"Out3\",\"Out4\",\"Out5\",\"Out6\"],\"side\":\"BOTTOM\"},\"type\":\"ConnectorPlacement.EquallySpacedRectSide\",\"uuid\":\"4528fa0d-8164-4e66-baa6-2a345765de4f\"}]},\"type\":\"ConnectorPlacement.EquallySpacedConnector\",\"uuid\":\"e6fb231a-8daf-4bfc-bdc1-9175fa7a2dfd\"}],\"packageUris\":[\"http://schema.mathworks.com/mf0/Connector/R2020b\"],\"version\":\"1.0\"}"
      mask Display: image('$imagefile')
  Relay : Relay  OnSwitchValue=1  OffSwitchValue=0  OnOutputValue=0  OffOutputValue=1
  "SOC Estimator " : BatteryEstimators/SOC Estimator (Coulomb Counting)  CurrentInputPartition=off  AH=10.52  Ts=1  DataType=Inherit: auto
      settings: LibrarySourceBlock=|
      | batt_sl_lib/Estimators/SOC Estimator
      | (Coulomb Counting)
  Simulink-PS Converter1 : nesl_utility/Simulink-PS Converter  PhysicalDomain=network_engine_domain  SubClassName=ps_input  LeftPortType=input  RightPortType=output  PseudoPeriodic=off  Frequencies=[]  NoiseDistribution=none  NoiseParameters=[]  Unit=1  AffineConversion=off  FilteringAndDerivatives=provide  SimscapeFilterOrder=1  InputFilterTimeConstant=0.001  UdotUserProvided=0
  Solver Configuration : nesl_utility/Solver Configuration  PhysicalDomain=network_engine_domain  SubClassName=solver  LeftPortType=input  RightPortType=generic  Tones=[]  Harmonics=[]  SimulateNoise=off  Profile=off  UseLocalSampling=off  EnableSwitchedLinearOptims=on  FrequencyDomain=off  UseCCode=off  RelTol=0.001  AbsTol=0.001  MinStep=1e-09  ToWorkspace=off  RevertToSquareIcSolve=off  NumHomotopyIterations=100  PhasorMode=off  PhasorModeNumHarmonics=1  ConsistencySolver=NEWTON_XTOL_AFTER_FTOL  CanonicalOrdering=CANONICAL  OptimizeIntermediates=OPTIMIZED  IndexReductionMethod=DerivativeReplacement  DoDC=off  ResidualTolerance=1e-09  ConsistencyTolSource=GLOBAL  ConsistencyAbsTol=0.001  ConsistencyRelTol=0.001  ConsistencyTolFactor=0.001  UseLocalSolver=off  LocalSolverChoice=NE_BACKWARD_EULER_ADVANCER  ResolveIndetEquations=on  FunctionEvalNumThread=1  LocalSolverSampleTime=0.001  DoFixedCost=off  MaxNonlinIter=3  MaxModeIter=2  ComputeImpulses=off  ImpulseIterations=2  LinearAlgebra=auto  LinearAlgebraNumThread=0  EquationFormulation=NE_TIME_EF  DelaysMemoryBudget=1024  AutomaticFiltering=on  FilteringTimeConstant=0.001  PartitionStorageMethod=AS_NEEDED  PartitionMemoryBudget=1024  PartitionMethod=ROBUST  MultibodyUseLocalSolver=off  MultibodyLocalSolverChoice=ODE1  MultibodyLocalSolverSampleTime=0.001
  Unit Delay : UnitDelay  InitialCondition=4.2
  Unit Delay1 : UnitDelay  InitialCondition=1
  Unit Delay2 : UnitDelay  SampleTime=-1
  AmbH : PMIOPort  Side=Right
  Current : Outport
  SOC : Outport  Port=2
  batteryTemperature : Outport  Port=3
  batteryVoltage : Outport  Port=4
  numCycles : Outport  Port=5
  soc_cell : Outport  Port=6
  socParallelAssembly : Outport  Port=7
  batteryCurrent : Outport  Port=8
  average_cell_voltage : Outport  Port=9
  wires:
  Project_Pack/1(batteryTemperature) -> batteryTemperature/1  "batteryTemperature"
  CC-CV Controller/1 -> ODPC/3(CC_CV_current)
  ODPC/1(output_current) -> Simulink-PS Converter1/1  "output_current"
  Gain1/1 -> CC-CV Controller/4
  Project_Pack/3(numCycles) -> numCycles/1
  Mean/1(y) -> average_cell_voltage/1, Unit Delay/1  "average_cell_voltage"
  Project_Pack/2(batteryVoltage) -> batteryVoltage/1
  Unit Delay1/1 -> ODPC/2(SOC), Relay/1
  Unit Delay2/1 -> ODPC/1(charging_enabled)
  Constant1/1 -> Gain/1, Gain1/1  "pack_C-rate"
  Unit Delay/1 -> CC-CV Controller/2
  Project_Pack/6(batteryCurrent) -> batteryCurrent/1
  Constant/1 -> "SOC Estimator "/2
  Project_Pack/4(socCell) -> soc_cell/1  "soc_cell"
  "SOC Estimator "/1 -> SOC/1, Unit Delay1/1  "SOC"
  Project_Pack/7(vParallelAssembly) -> Mean/1(u)
  PS-Simulink Converter/1 -> Current/1, "SOC Estimator "/1
  Gain/1 -> CC-CV Controller/3
  Relay/1 -> Unit Delay2/1, CC-CV Controller/1  "charging_enabled"
  Project_Pack/5(socParallelAssembly) -> socParallelAssembly/1
  connections:
  Project_Pack/RConn1 -- AmbH/RConn1
  Controlled Current Source/LConn1 -- Project_Pack/LConn1
  Simulink-PS Converter1/RConn1 -- Controlled Current Source/RConn1
  Project_Pack/RConn2 -- Solver Configuration/RConn1 -- Current Sensor/LConn1 -- Electrical Reference/LConn1
  Current Sensor/RConn1 -- PS-Simulink Converter/LConn1
  Current Sensor/RConn2 -- Controlled Current Source/RConn2

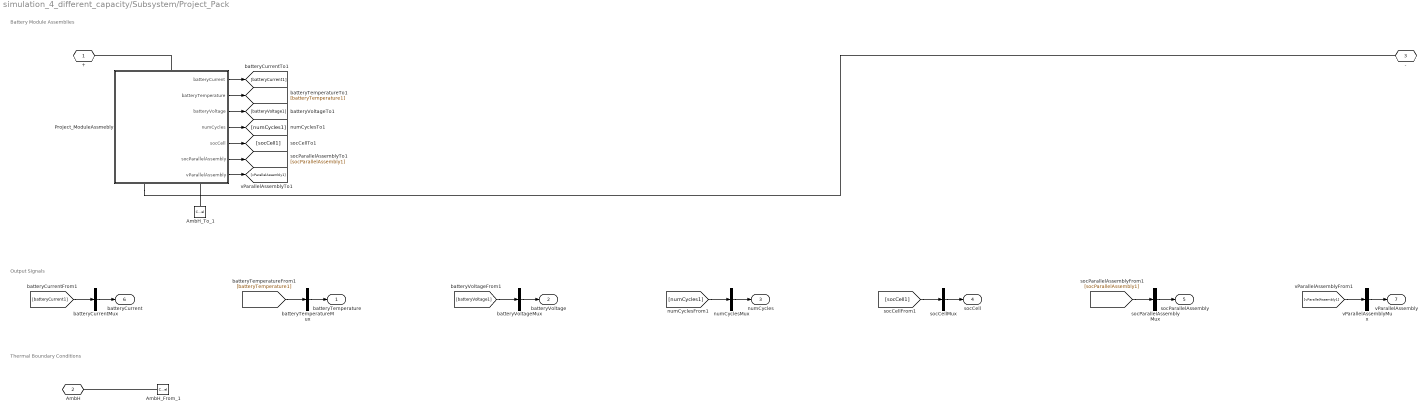
== system simulation_4_different_capacity/Subsystem/Project_Pack ==
  note: Thermal Boundary Conditions
  note: Output Signals
  note: Battery Module Assemblies
  AmbH_From_1 : ConnectionLabel  Label=ambH_1
  AmbH_To_1 : ConnectionLabel  Label=ambH_1
  Project_ModuleAssmebly : Subsystem  LoadFcn=battery_builder_rtmsupport('loadfcn',gcbh);
      settings: CopyFcn=battery_builder_rtmsupport('copyfcn',gcbh);  PreCopyFcn=battery_builder_rtmsupport('precopyfcn',gcbh);  PreDeleteFcn=battery_builder_rtmsupport('predeletefcn',gcbh);  PortSchema="{\"entries\":[{\"content\":{\"sides\":[{\"content\":{\"connectorIds\":[\"LConn1\"]},\"type\":\"ConnectorPlacement.EquallySpacedRectSide\",\"uuid\":\"76c6f046-db8e-4015-a922-00ba973faf16\"},{\"content\":{\"connectorIds\":[\"RConn1\",\"RConn2\"],\"side\":\"RIGHT\"},\"type\":\"ConnectorPlacement.EquallySpacedRectSide\",\"uuid\":\"59fdee5c-a6f4-4b44-aa6e-82d2d9418fce\"},{\"content\":{\"side\":\"TOP\"},\"type\":\"ConnectorPlacement.EquallySpacedRectSide\",\"uuid\":\"84b83595-cc1f-46da-a2b0-c16634a6daab\"},{\"content\":{\"connectorIds\":[\"Out1\",\"Out2\",\"Out3\",\"Out4\",\"Out5\",\"Out6\",\"Out7\"],\"side\":\"BOTTOM\"},\"type\":\"ConnectorPlacement.EquallySpacedRectSide\",\"uuid\":\"391f6102-8f79-4306-a331-0bb83eeeb4a2\"}]},\"type\":\"ConnectorPlacement.EquallySpacedConnector\",\"uuid\":\"e6fb231a-8daf-4bfc-bdc1-9175fa7a2dfd\"}],\"packageUris\":[\"http://schema.mathworks.com/mf0/Connector/R2020b\"],\"version\":\"1.0\"}"
      mask Display: image('$imagefile')
  batteryCurrentMux : Mux  Inputs=1
  batteryTemperatureMux : Mux  Inputs=1
  batteryVoltageMux : Mux  Inputs=1
  numCyclesMux : Mux  Inputs=1
  socCellMux : Mux  Inputs=1
  socParallelAssemblyMux : Mux  Inputs=1
  vParallelAssemblyMux : Mux  Inputs=1
  + : PMIOPort  Side=Left
  AmbH : PMIOPort  Port=2  Side=Right  ConnectionType=Connection: foundation.thermal.thermal
  - : PMIOPort  Port=3  Side=Right
  batteryTemperature : Outport
  batteryVoltage : Outport  Port=2
  numCycles : Outport  Port=3
  socCell : Outport  Port=4
  socParallelAssembly : Outport  Port=5
  batteryCurrent : Outport  Port=6
  vParallelAssembly : Outport  Port=7
  wires:
  [vParallelAssembly1] -> vParallelAssemblyMux/1
  vParallelAssemblyMux/1 -> vParallelAssembly/1
  Project_ModuleAssmebly/7(vParallelAssembly) -> [vParallelAssembly1]
  [socParallelAssembly1] -> socParallelAssemblyMux/1
  socParallelAssemblyMux/1 -> socParallelAssembly/1
  Project_ModuleAssmebly/6(socParallelAssembly) -> [socParallelAssembly1]
  [socCell1] -> socCellMux/1
  socCellMux/1 -> socCell/1
  Project_ModuleAssmebly/5(socCell) -> [socCell1]
  [numCycles1] -> numCyclesMux/1
  numCyclesMux/1 -> numCycles/1
  Project_ModuleAssmebly/4(numCycles) -> [numCycles1]
  [batteryVoltage1] -> batteryVoltageMux/1
  batteryVoltageMux/1 -> batteryVoltage/1
  Project_ModuleAssmebly/3(batteryVoltage) -> [batteryVoltage1]
  [batteryTemperature1] -> batteryTemperatureMux/1
  batteryTemperatureMux/1 -> batteryTemperature/1
  Project_ModuleAssmebly/2(batteryTemperature) -> [batteryTemperature1]
  [batteryCurrent1] -> batteryCurrentMux/1
  batteryCurrentMux/1 -> batteryCurrent/1
  Project_ModuleAssmebly/1(batteryCurrent) -> [batteryCurrent1]
  connections:
  AmbH_From_1/LConn1 -- AmbH/RConn1
  AmbH_To_1/LConn1 -- Project_ModuleAssmebly/RConn2
  Project_ModuleAssmebly/RConn1 -- -/RConn1
  Project_ModuleAssmebly/LConn1 -- +/RConn1

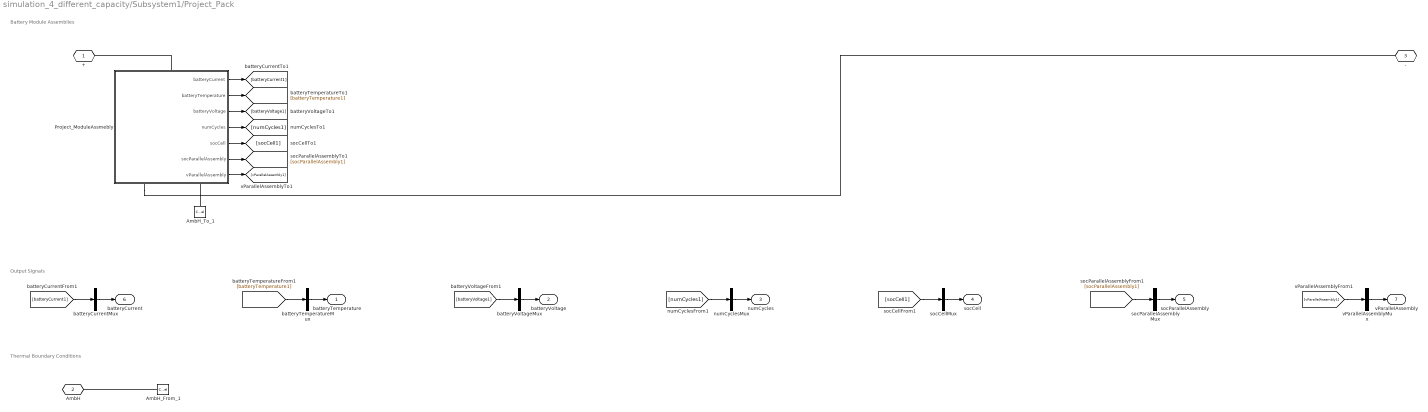
== system simulation_4_different_capacity/Subsystem1/Project_Pack ==
  note: Thermal Boundary Conditions
  note: Output Signals
  note: Battery Module Assemblies
  AmbH_From_1 : ConnectionLabel  Label=ambH_1
  AmbH_To_1 : ConnectionLabel  Label=ambH_1
  Project_ModuleAssmebly : Subsystem  LoadFcn=battery_builder_rtmsupport('loadfcn',gcbh);
      settings: CopyFcn=battery_builder_rtmsupport('copyfcn',gcbh);  PreCopyFcn=battery_builder_rtmsupport('precopyfcn',gcbh);  PreDeleteFcn=battery_builder_rtmsupport('predeletefcn',gcbh);  PortSchema="{\"entries\":[{\"content\":{\"sides\":[{\"content\":{\"connectorIds\":[\"LConn1\"]},\"type\":\"ConnectorPlacement.EquallySpacedRectSide\",\"uuid\":\"76c6f046-db8e-4015-a922-00ba973faf16\"},{\"content\":{\"connectorIds\":[\"RConn1\",\"RConn2\"],\"side\":\"RIGHT\"},\"type\":\"ConnectorPlacement.EquallySpacedRectSide\",\"uuid\":\"59fdee5c-a6f4-4b44-aa6e-82d2d9418fce\"},{\"content\":{\"side\":\"TOP\"},\"type\":\"ConnectorPlacement.EquallySpacedRectSide\",\"uuid\":\"84b83595-cc1f-46da-a2b0-c16634a6daab\"},{\"content\":{\"connectorIds\":[\"Out1\",\"Out2\",\"Out3\",\"Out4\",\"Out5\",\"Out6\",\"Out7\"],\"side\":\"BOTTOM\"},\"type\":\"ConnectorPlacement.EquallySpacedRectSide\",\"uuid\":\"391f6102-8f79-4306-a331-0bb83eeeb4a2\"}]},\"type\":\"ConnectorPlacement.EquallySpacedConnector\",\"uuid\":\"e6fb231a-8daf-4bfc-bdc1-9175fa7a2dfd\"}],\"packageUris\":[\"http://schema.mathworks.com/mf0/Connector/R2020b\"],\"version\":\"1.0\"}"
      mask Display: image('$imagefile')
  batteryCurrentMux : Mux  Inputs=1
  batteryTemperatureMux : Mux  Inputs=1
  batteryVoltageMux : Mux  Inputs=1
  numCyclesMux : Mux  Inputs=1
  socCellMux : Mux  Inputs=1
  socParallelAssemblyMux : Mux  Inputs=1
  vParallelAssemblyMux : Mux  Inputs=1
  + : PMIOPort  Side=Left
  AmbH : PMIOPort  Port=2  Side=Right  ConnectionType=Connection: foundation.thermal.thermal
  - : PMIOPort  Port=3  Side=Right
  batteryTemperature : Outport
  batteryVoltage : Outport  Port=2
  numCycles : Outport  Port=3
  socCell : Outport  Port=4
  socParallelAssembly : Outport  Port=5
  batteryCurrent : Outport  Port=6
  vParallelAssembly : Outport  Port=7
  wires:
  [vParallelAssembly1] -> vParallelAssemblyMux/1
  vParallelAssemblyMux/1 -> vParallelAssembly/1
  Project_ModuleAssmebly/7(vParallelAssembly) -> [vParallelAssembly1]
  [socParallelAssembly1] -> socParallelAssemblyMux/1
  socParallelAssemblyMux/1 -> socParallelAssembly/1
  Project_ModuleAssmebly/6(socParallelAssembly) -> [socParallelAssembly1]
  [socCell1] -> socCellMux/1
  socCellMux/1 -> socCell/1
  Project_ModuleAssmebly/5(socCell) -> [socCell1]
  [numCycles1] -> numCyclesMux/1
  numCyclesMux/1 -> numCycles/1
  Project_ModuleAssmebly/4(numCycles) -> [numCycles1]
  [batteryVoltage1] -> batteryVoltageMux/1
  batteryVoltageMux/1 -> batteryVoltage/1
  Project_ModuleAssmebly/3(batteryVoltage) -> [batteryVoltage1]
  [batteryTemperature1] -> batteryTemperatureMux/1
  batteryTemperatureMux/1 -> batteryTemperature/1
  Project_ModuleAssmebly/2(batteryTemperature) -> [batteryTemperature1]
  [batteryCurrent1] -> batteryCurrentMux/1
  batteryCurrentMux/1 -> batteryCurrent/1
  Project_ModuleAssmebly/1(batteryCurrent) -> [batteryCurrent1]
  connections:
  AmbH_From_1/LConn1 -- AmbH/RConn1
  AmbH_To_1/LConn1 -- Project_ModuleAssmebly/RConn2
  Project_ModuleAssmebly/RConn1 -- -/RConn1
  Project_ModuleAssmebly/LConn1 -- +/RConn1
